simulink subsystem "CrossProductMatrix"  (R2024b)
settings: Solver=VariableStepAuto  StartTime=0.0  StopTime=10.0  RelTol=1e-3
settings Model: Creator=marco  LastModifiedBy=ferru

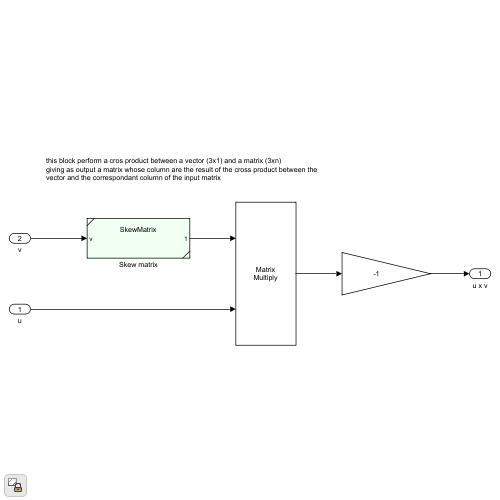
[thumbnail: Simulink's stored preview of the top-level diagram]
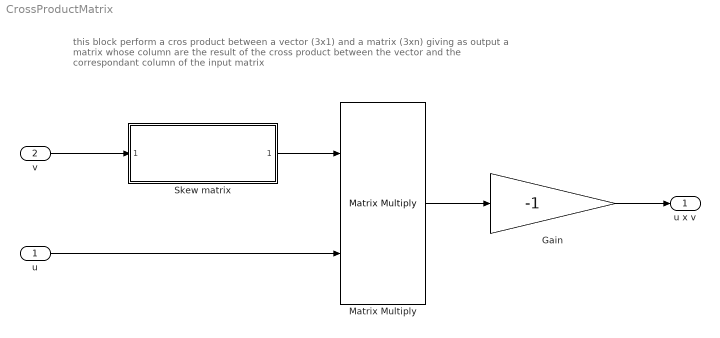
== system CrossProductMatrix ==
  note: this block perform a cros product between a vector (3x1) and a matrix (3xn)
      | giving as output a matrix whose column are the result of the cross product between the vector and the correspondant column of the input matrix
  u : Inport
  v : Inport  Port=2
  Gain : Gain  Gain=-1
  Matrix Multiply : Product  Multiplication=Matrix(*)
  Skew matrix : Subsystem  ReferencedSubsystem=SkewMatrix
  u x v : Outport
  wires:
  v/1 -> Skew matrix/1
  u/1 -> Matrix Multiply/2
  Skew matrix/1 -> Matrix Multiply/1
  Matrix Multiply/1 -> Gain/1
  Gain/1 -> u x v/1
